simulink model "u2i_4"  (R2024a)
settings: Solver=VariableStepAuto  StartTime=0.0  StopTime=0.1  RelTol=1e-3
libraries: fl_lib x107, ee_lib x90, nesl_utility x40
(part 1 of 9)
settings Model: Creator=ltnbda  LastModifiedBy=dbagn
settings RTWCC: GPUComputeCapability=3.5

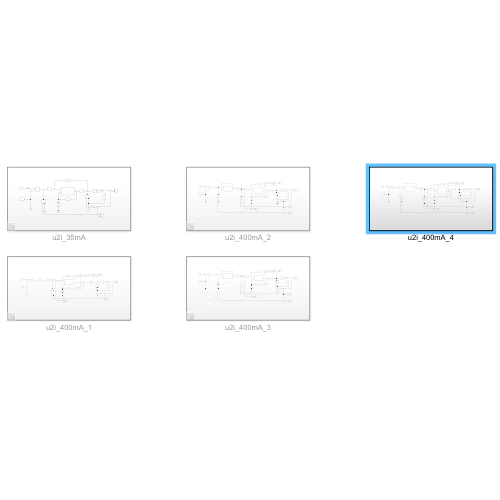
[thumbnail: Simulink's stored preview of the top-level diagram]
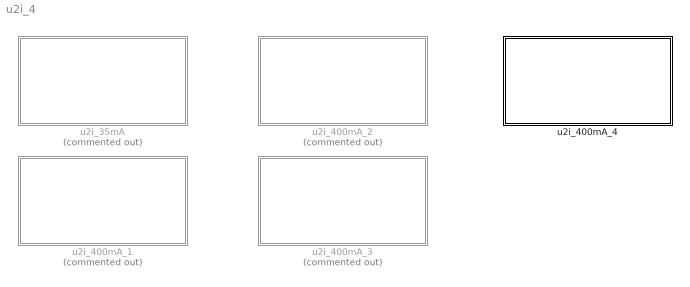
== system u2i_4 ==
  u2i_35mA : Subsystem  Commented=on
  u2i_400mA_1 : Subsystem  Commented=on
  u2i_400mA_2 : Subsystem  Commented=on
  u2i_400mA_3 : Subsystem  Commented=on
  u2i_400mA_4 : Subsystem

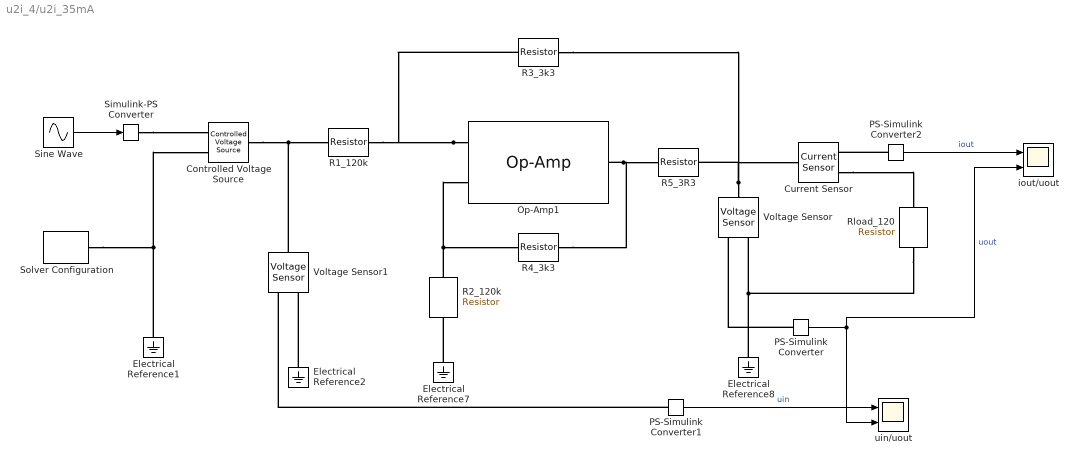
== system u2i_4/u2i_35mA ==
  Controlled Voltage Source : fl_lib/Electrical/Electrical Sources/Controlled Voltage Source
  Current Sensor : fl_lib/Electrical/Electrical Sensors/Current Sensor
  Electrical Reference{1..2,7..8} (4 alike) : fl_lib/Electrical/Electrical Elements/Electrical Reference
  Op-Amp1 : fl_lib/Electrical/Electrical Elements/Op-Amp  outI_specify=off  outI_priority=None  outI=0 A  outI_nominal_specify=off  outI_nominal_value=1  outI_nominal_unit=A
  PS-Simulink Converter : nesl_utility/PS-Simulink Converter  PhysicalDomain=network_engine_domain  SubClassName=ps_output  LeftPortType=input  RightPortType=output  PseudoPeriodic=off  Frequencies=[]  VectorFormat=1-D array  Unit=V  AffineConversion=off
  PS-Simulink Converter1 : nesl_utility/PS-Simulink Converter  PhysicalDomain=network_engine_domain  SubClassName=ps_output  LeftPortType=input  RightPortType=output  PseudoPeriodic=off  Frequencies=[]  VectorFormat=1-D array  Unit=V  AffineConversion=off
  PS-Simulink Converter2 : nesl_utility/PS-Simulink Converter  PhysicalDomain=network_engine_domain  SubClassName=ps_output  LeftPortType=input  RightPortType=output  PseudoPeriodic=off  Frequencies=[]  VectorFormat=1-D array  Unit=A  AffineConversion=off
  R1_120k : fl_lib/Electrical/Electrical Elements/Resistor  R=120e3 Ohm  i_specify=off  i_priority=None  i=0 A  i_nominal_specify=off  i_nominal_value=1  i_nominal_unit=A  v_specify=off  v_priority=None  v=0 V  v_nominal_specify=off  v_nominal_value=1  v_nominal_unit=V
  R2_120k : fl_lib/Electrical/Electrical Elements/Resistor  R=120e3 Ohm  i_specify=off  i_priority=None  i=0 A  i_nominal_specify=off  i_nominal_value=1  i_nominal_unit=A  v_specify=off  v_priority=None  v=0 V  v_nominal_specify=off  v_nominal_value=1  v_nominal_unit=V
  R3_3k3 : fl_lib/Electrical/Electrical Elements/Resistor  R=3.3e3 Ohm  i_specify=off  i_priority=None  i=0 A  i_nominal_specify=off  i_nominal_value=1  i_nominal_unit=A  v_specify=off  v_priority=None  v=0 V  v_nominal_specify=off  v_nominal_value=1  v_nominal_unit=V
  R4_3k3 : fl_lib/Electrical/Electrical Elements/Resistor  R=3.3e3 Ohm  i_specify=off  i_priority=None  i=0 A  i_nominal_specify=off  i_nominal_value=1  i_nominal_unit=A  v_specify=off  v_priority=None  v=0 V  v_nominal_specify=off  v_nominal_value=1  v_nominal_unit=V
  R5_3R3 : fl_lib/Electrical/Electrical Elements/Resistor  R=3.3 Ohm  i_specify=off  i_priority=None  i=0 A  i_nominal_specify=off  i_nominal_value=1  i_nominal_unit=A  v_specify=off  v_priority=None  v=0 V  v_nominal_specify=off  v_nominal_value=1  v_nominal_unit=V
  Rload_120 : fl_lib/Electrical/Electrical Elements/Resistor  R=12 Ohm  i_specify=off  i_priority=None  i=0 A  i_nominal_specify=off  i_nominal_value=1  i_nominal_unit=A  v_specify=off  v_priority=None  v=0 V  v_nominal_specify=off  v_nominal_value=1  v_nominal_unit=V
  Simulink-PS Converter : nesl_utility/Simulink-PS Converter  PhysicalDomain=network_engine_domain  SubClassName=ps_input  LeftPortType=input  RightPortType=output  PseudoPeriodic=off  Frequencies=[]  NoiseDistribution=none  NoiseParameters=[]  Unit=V  AffineConversion=off  FilteringAndDerivatives=provide  SimscapeFilterOrder=1  InputFilterTimeConstant=0.001  UdotUserProvided=0
  Sine Wave : Sin  Amplitude=2  Frequency=2*pi*50  SampleTime=0
  Solver Configuration : nesl_utility/Solver Configuration  PhysicalDomain=network_engine_domain  SubClassName=solver  LeftPortType=input  RightPortType=generic  Tones=[]  Harmonics=[]  SimulateNoise=off  Profile=off  UseLocalSampling=off  EnableSwitchedLinearOptims=on  FrequencyDomain=off  UseCCode=off  RelTol=0.001  AbsTol=0.001  MinStep=1e-09  ToWorkspace=off  RevertToSquareIcSolve=off  NumHomotopyIterations=100  PhasorMode=off  PhasorModeNumHarmonics=1  ConsistencySolver=NEWTON_XTOL_AFTER_FTOL  IndexReductionMethod=DerivativeReplacement  DoDC=on  ResidualTolerance=1e-09  ConsistencyTolSource=GLOBAL  ConsistencyAbsTol=0.001  ConsistencyRelTol=0.001  ConsistencyTolFactor=0.001  UseLocalSolver=on  LocalSolverChoice=NE_BACKWARD_EULER_ADVANCER  ResolveIndetEquations=on  FunctionEvalNumThread=1  LocalSolverSampleTime=1e-6  DoFixedCost=on  MaxNonlinIter=3  MaxModeIter=2  ComputeImpulses=off  ImpulseIterations=2  LinearAlgebra=auto  LinearAlgebraNumThread=0  EquationFormulation=NE_TIME_EF  DelaysMemoryBudget=1024  AutomaticFiltering=on  FilteringTimeConstant=0.001  PartitionStorageMethod=AS_NEEDED  PartitionMemoryBudget=1024  PartitionMethod=ROBUST  MultibodyUseLocalSolver=off  MultibodyLocalSolverChoice=ODE1  MultibodyLocalSolverSampleTime=0.001
  Voltage Sensor : fl_lib/Electrical/Electrical Sensors/Voltage Sensor
  Voltage Sensor1 : fl_lib/Electrical/Electrical Sensors/Voltage Sensor
  iout/uout : Scope  NumInputPorts=2
  uin/uout : Scope  NumInputPorts=2
  wires:
  PS-Simulink Converter2/1 -> iout/uout/1  "iout"
  PS-Simulink Converter1/1 -> uin/uout/1  "uin"
  PS-Simulink Converter/1 -> uin/uout/2, iout/uout/2  "uout"
  Sine Wave/1 -> Simulink-PS Converter/1
  connections:
  Voltage Sensor/LConn1 -- Current Sensor/LConn1 -- R3_3k3/RConn1 -- R5_3R3/RConn1
  Op-Amp1/RConn1 -- R5_3R3/LConn1 -- R4_3k3/RConn1
  R2_120k/LConn1 -- R4_3k3/LConn1 -- Op-Amp1/LConn2
  Electrical Reference8/LConn1 -- Voltage Sensor/RConn2 -- Rload_120/RConn1
  Electrical Reference1/LConn1 -- Solver Configuration/RConn1 -- Controlled Voltage Source/RConn2
  Op-Amp1/LConn1 -- R3_3k3/LConn1 -- R1_120k/RConn1
  PS-Simulink Converter/LConn1 -- Voltage Sensor/RConn1
  Electrical Reference7/LConn1 -- R2_120k/RConn1
  Simulink-PS Converter/RConn1 -- Controlled Voltage Source/RConn1
  Electrical Reference2/LConn1 -- Voltage Sensor1/RConn2
  Controlled Voltage Source/LConn1 -- Voltage Sensor1/LConn1 -- R1_120k/LConn1
  PS-Simulink Converter2/LConn1 -- Current Sensor/RConn1
  Current Sensor/RConn2 -- Rload_120/LConn1
  PS-Simulink Converter1/LConn1 -- Voltage Sensor1/RConn1

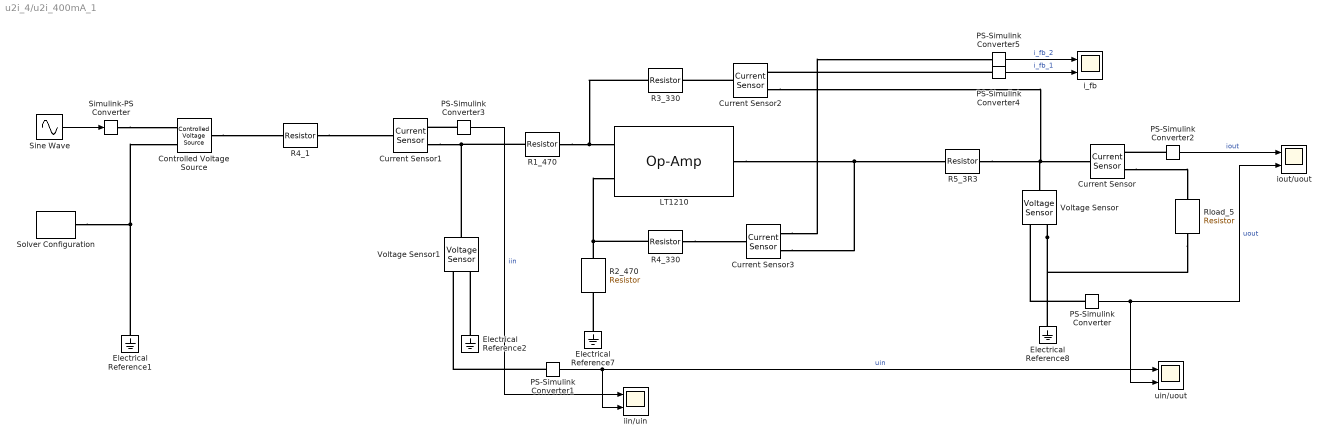
== system u2i_4/u2i_400mA_1 ==
  Controlled Voltage Source : fl_lib/Electrical/Electrical Sources/Controlled Voltage Source
  Current Sensor{,1..3} (4 alike) : fl_lib/Electrical/Electrical Sensors/Current Sensor
  Electrical Reference{1..2,7..8} (4 alike) : fl_lib/Electrical/Electrical Elements/Electrical Reference
  LT1210 : fl_lib/Electrical/Electrical Elements/Op-Amp  outI_specify=off  outI_priority=None  outI=0 A  outI_nominal_specify=off  outI_nominal_value=1  outI_nominal_unit=A
  PS-Simulink Converter : nesl_utility/PS-Simulink Converter  PhysicalDomain=network_engine_domain  SubClassName=ps_output  LeftPortType=input  RightPortType=output  PseudoPeriodic=off  Frequencies=[]  VectorFormat=1-D array  Unit=V  AffineConversion=off
  PS-Simulink Converter1 : nesl_utility/PS-Simulink Converter  PhysicalDomain=network_engine_domain  SubClassName=ps_output  LeftPortType=input  RightPortType=output  PseudoPeriodic=off  Frequencies=[]  VectorFormat=1-D array  Unit=V  AffineConversion=off
  PS-Simulink Converter{2..5} (4 alike) : nesl_utility/PS-Simulink Converter  PhysicalDomain=network_engine_domain  SubClassName=ps_output  LeftPortType=input  RightPortType=output  PseudoPeriodic=off  Frequencies=[]  VectorFormat=1-D array  Unit=A  AffineConversion=off
  R1_470 : fl_lib/Electrical/Electrical Elements/Resistor  R=470 Ohm  i_specify=off  i_priority=None  i=0 A  i_nominal_specify=off  i_nominal_value=1  i_nominal_unit=A  v_specify=off  v_priority=None  v=0 V  v_nominal_specify=off  v_nominal_value=1  v_nominal_unit=V
  R2_470 : fl_lib/Electrical/Electrical Elements/Resistor  R=470 Ohm  i_specify=off  i_priority=None  i=0 A  i_nominal_specify=off  i_nominal_value=1  i_nominal_unit=A  v_specify=off  v_priority=None  v=0 V  v_nominal_specify=off  v_nominal_value=1  v_nominal_unit=V
  R3_330 : fl_lib/Electrical/Electrical Elements/Resistor  R=330 Ohm  i_specify=off  i_priority=None  i=0 A  i_nominal_specify=off  i_nominal_value=1  i_nominal_unit=A  v_specify=off  v_priority=None  v=0 V  v_nominal_specify=off  v_nominal_value=1  v_nominal_unit=V
  R4_1 : fl_lib/Electrical/Electrical Elements/Resistor  R=0 Ohm  i_specify=off  i_priority=None  i=0 A  i_nominal_specify=off  i_nominal_value=1  i_nominal_unit=A  v_specify=off  v_priority=None  v=0 V  v_nominal_specify=off  v_nominal_value=1  v_nominal_unit=V
  R4_330 : fl_lib/Electrical/Electrical Elements/Resistor  R=330 Ohm  i_specify=off  i_priority=None  i=0 A  i_nominal_specify=off  i_nominal_value=1  i_nominal_unit=A  v_specify=off  v_priority=None  v=0 V  v_nominal_specify=off  v_nominal_value=1  v_nominal_unit=V
  R5_3R3 : fl_lib/Electrical/Electrical Elements/Resistor  R=3.3 Ohm  i_specify=off  i_priority=None  i=0 A  i_nominal_specify=off  i_nominal_value=1  i_nominal_unit=A  v_specify=off  v_priority=None  v=0 V  v_nominal_specify=off  v_nominal_value=1  v_nominal_unit=V
  Rload_5 : fl_lib/Electrical/Electrical Elements/Resistor  R=10 Ohm  i_specify=off  i_priority=None  i=0 A  i_nominal_specify=off  i_nominal_value=1  i_nominal_unit=A  v_specify=off  v_priority=None  v=0 V  v_nominal_specify=off  v_nominal_value=1  v_nominal_unit=V
  Simulink-PS Converter : nesl_utility/Simulink-PS Converter  PhysicalDomain=network_engine_domain  SubClassName=ps_input  LeftPortType=input  RightPortType=output  PseudoPeriodic=off  Frequencies=[]  NoiseDistribution=none  NoiseParameters=[]  Unit=V  AffineConversion=off  FilteringAndDerivatives=provide  SimscapeFilterOrder=1  InputFilterTimeConstant=0.001  UdotUserProvided=0
  Sine Wave : Sin  Amplitude=2  Frequency=2*pi*50  SampleTime=0
  Solver Configuration : nesl_utility/Solver Configuration  PhysicalDomain=network_engine_domain  SubClassName=solver  LeftPortType=input  RightPortType=generic  Tones=[]  Harmonics=[]  SimulateNoise=off  Profile=off  UseLocalSampling=off  EnableSwitchedLinearOptims=on  FrequencyDomain=off  UseCCode=off  RelTol=0.001  AbsTol=0.001  MinStep=1e-09  ToWorkspace=off  RevertToSquareIcSolve=off  NumHomotopyIterations=100  PhasorMode=off  PhasorModeNumHarmonics=1  ConsistencySolver=NEWTON_XTOL_AFTER_FTOL  IndexReductionMethod=DerivativeReplacement  DoDC=on  ResidualTolerance=1e-09  ConsistencyTolSource=GLOBAL  ConsistencyAbsTol=0.001  ConsistencyRelTol=0.001  ConsistencyTolFactor=0.001  UseLocalSolver=on  LocalSolverChoice=NE_BACKWARD_EULER_ADVANCER  ResolveIndetEquations=on  FunctionEvalNumThread=1  LocalSolverSampleTime=1e-6  DoFixedCost=on  MaxNonlinIter=3  MaxModeIter=2  ComputeImpulses=off  ImpulseIterations=2  LinearAlgebra=auto  LinearAlgebraNumThread=0  EquationFormulation=NE_TIME_EF  DelaysMemoryBudget=1024  AutomaticFiltering=on  FilteringTimeConstant=0.001  PartitionStorageMethod=AS_NEEDED  PartitionMemoryBudget=1024  PartitionMethod=ROBUST  MultibodyUseLocalSolver=off  MultibodyLocalSolverChoice=ODE1  MultibodyLocalSolverSampleTime=0.001
  Voltage Sensor : fl_lib/Electrical/Electrical Sensors/Voltage Sensor
  Voltage Sensor1 : fl_lib/Electrical/Electrical Sensors/Voltage Sensor
  i_fb : Scope  NumInputPorts=2
  iin/uin : Scope  NumInputPorts=2
  iout/uout : Scope  NumInputPorts=2
  uin/uout : Scope  NumInputPorts=2
  wires:
  Sine Wave/1 -> Simulink-PS Converter/1
  PS-Simulink Converter/1 -> iout/uout/2, uin/uout/2  "uout"
  PS-Simulink Converter1/1 -> uin/uout/1, iin/uin/2  "uin"
  PS-Simulink Converter2/1 -> iout/uout/1  "iout"
  PS-Simulink Converter3/1 -> iin/uin/1  "iin"
  PS-Simulink Converter4/1 -> i_fb/2  "i_fb_1"
  PS-Simulink Converter5/1 -> i_fb/1  "i_fb_2"
  connections:
  PS-Simulink Converter1/LConn1 -- Voltage Sensor1/RConn1
  Current Sensor/RConn2 -- Rload_5/LConn1
  PS-Simulink Converter2/LConn1 -- Current Sensor/RConn1
  Voltage Sensor1/LConn1 -- R1_470/LConn1 -- Current Sensor1/RConn2
  Electrical Reference2/LConn1 -- Voltage Sensor1/RConn2
  Simulink-PS Converter/RConn1 -- Controlled Voltage Source/RConn1
  Electrical Reference7/LConn1 -- R2_470/RConn1
  PS-Simulink Converter/LConn1 -- Voltage Sensor/RConn1
  Solver Configuration/RConn1 -- Controlled Voltage Source/RConn2 -- Electrical Reference1/LConn1
  Voltage Sensor/RConn2 -- Electrical Reference8/LConn1 -- Rload_5/RConn1
  R2_470/LConn1 -- LT1210/LConn2 -- R4_330/LConn1
  LT1210/RConn1 -- Current Sensor3/RConn2 -- R5_3R3/LConn1
  PS-Simulink Converter3/LConn1 -- Current Sensor1/RConn1
  R1_470/RConn1 -- R3_330/LConn1 -- LT1210/LConn1
  R5_3R3/RConn1 -- Current Sensor2/RConn2 -- Voltage Sensor/LConn1 -- Current Sensor/LConn1
  R4_1/RConn1 -- Current Sensor1/LConn1
  Current Sensor2/LConn1 -- R3_330/RConn1
  PS-Simulink Converter4/LConn1 -- Current Sensor2/RConn1
  R4_330/RConn1 -- Current Sensor3/LConn1
  Current Sensor3/RConn1 -- PS-Simulink Converter5/LConn1
  Controlled Voltage Source/LConn1 -- R4_1/LConn1

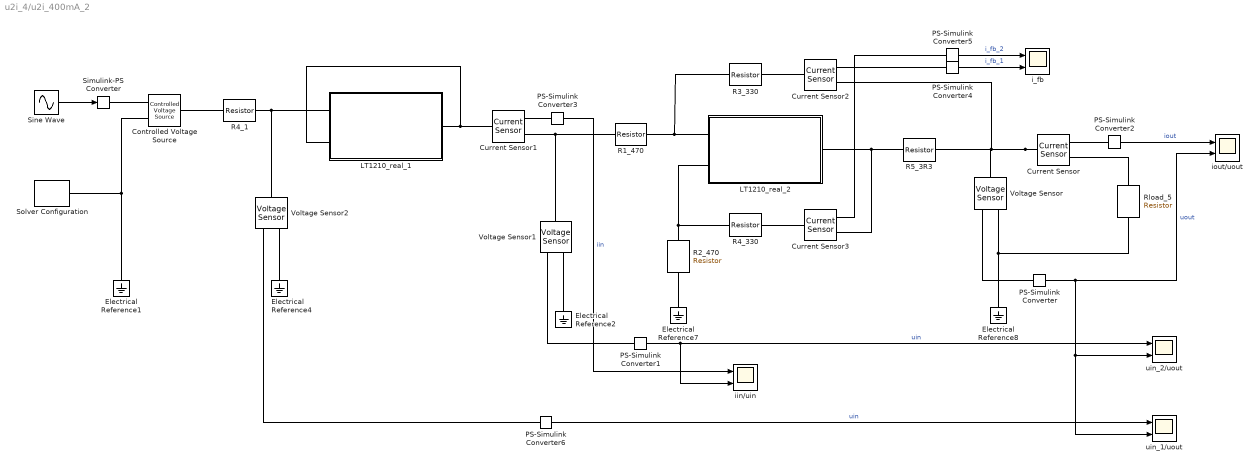
== system u2i_4/u2i_400mA_2 ==
  Controlled Voltage Source : fl_lib/Electrical/Electrical Sources/Controlled Voltage Source
  Current Sensor{,1..3} (4 alike) : fl_lib/Electrical/Electrical Sensors/Current Sensor
  Electrical Reference{1..2,4,7..8} (5 alike) : fl_lib/Electrical/Electrical Elements/Electrical Reference
  LT1210_real_1 : Subsystem
  LT1210_real_2 : Subsystem
  PS-Simulink Converter : nesl_utility/PS-Simulink Converter  PhysicalDomain=network_engine_domain  SubClassName=ps_output  LeftPortType=input  RightPortType=output  PseudoPeriodic=off  Frequencies=[]  VectorFormat=1-D array  Unit=V  AffineConversion=off
  PS-Simulink Converter1 : nesl_utility/PS-Simulink Converter  PhysicalDomain=network_engine_domain  SubClassName=ps_output  LeftPortType=input  RightPortType=output  PseudoPeriodic=off  Frequencies=[]  VectorFormat=1-D array  Unit=V  AffineConversion=off
  PS-Simulink Converter{2..5} (4 alike) : nesl_utility/PS-Simulink Converter  PhysicalDomain=network_engine_domain  SubClassName=ps_output  LeftPortType=input  RightPortType=output  PseudoPeriodic=off  Frequencies=[]  VectorFormat=1-D array  Unit=A  AffineConversion=off
  PS-Simulink Converter6 : nesl_utility/PS-Simulink Converter  PhysicalDomain=network_engine_domain  SubClassName=ps_output  LeftPortType=input  RightPortType=output  PseudoPeriodic=off  Frequencies=[]  VectorFormat=1-D array  Unit=V  AffineConversion=off
  R1_470 : fl_lib/Electrical/Electrical Elements/Resistor  R=470 Ohm  i_specify=off  i_priority=None  i=0 A  i_nominal_specify=off  i_nominal_value=1  i_nominal_unit=A  v_specify=off  v_priority=None  v=0 V  v_nominal_specify=off  v_nominal_value=1  v_nominal_unit=V
  R2_470 : fl_lib/Electrical/Electrical Elements/Resistor  R=470 Ohm  i_specify=off  i_priority=None  i=0 A  i_nominal_specify=off  i_nominal_value=1  i_nominal_unit=A  v_specify=off  v_priority=None  v=0 V  v_nominal_specify=off  v_nominal_value=1  v_nominal_unit=V
  R3_330 : fl_lib/Electrical/Electrical Elements/Resistor  R=330 Ohm  i_specify=off  i_priority=None  i=0 A  i_nominal_specify=off  i_nominal_value=1  i_nominal_unit=A  v_specify=off  v_priority=None  v=0 V  v_nominal_specify=off  v_nominal_value=1  v_nominal_unit=V
  R4_1 : fl_lib/Electrical/Electrical Elements/Resistor  R=1e3 Ohm  i_specify=off  i_priority=None  i=0 A  i_nominal_specify=off  i_nominal_value=1  i_nominal_unit=A  v_specify=off  v_priority=None  v=0 V  v_nominal_specify=off  v_nominal_value=1  v_nominal_unit=V
  R4_330 : fl_lib/Electrical/Electrical Elements/Resistor  R=330 Ohm  i_specify=off  i_priority=None  i=0 A  i_nominal_specify=off  i_nominal_value=1  i_nominal_unit=A  v_specify=off  v_priority=None  v=0 V  v_nominal_specify=off  v_nominal_value=1  v_nominal_unit=V
  R5_3R3 : fl_lib/Electrical/Electrical Elements/Resistor  R=3.3 Ohm  i_specify=off  i_priority=None  i=0 A  i_nominal_specify=off  i_nominal_value=1  i_nominal_unit=A  v_specify=off  v_priority=None  v=0 V  v_nominal_specify=off  v_nominal_value=1  v_nominal_unit=V
  Rload_5 : fl_lib/Electrical/Electrical Elements/Resistor  R=10 Ohm  i_specify=off  i_priority=None  i=0 A  i_nominal_specify=off  i_nominal_value=1  i_nominal_unit=A  v_specify=off  v_priority=None  v=0 V  v_nominal_specify=off  v_nominal_value=1  v_nominal_unit=V
  Simulink-PS Converter : nesl_utility/Simulink-PS Converter  PhysicalDomain=network_engine_domain  SubClassName=ps_input  LeftPortType=input  RightPortType=output  PseudoPeriodic=off  Frequencies=[]  NoiseDistribution=none  NoiseParameters=[]  Unit=V  AffineConversion=off  FilteringAndDerivatives=provide  SimscapeFilterOrder=1  InputFilterTimeConstant=0.001  UdotUserProvided=0
  Sine Wave : Sin  Amplitude=2  Frequency=2*pi*50  SampleTime=0
  Solver Configuration : nesl_utility/Solver Configuration  PhysicalDomain=network_engine_domain  SubClassName=solver  LeftPortType=input  RightPortType=generic  Tones=[]  Harmonics=[]  SimulateNoise=off  Profile=off  UseLocalSampling=off  EnableSwitchedLinearOptims=on  FrequencyDomain=off  UseCCode=off  RelTol=0.001  AbsTol=0.001  MinStep=1e-09  ToWorkspace=off  RevertToSquareIcSolve=off  NumHomotopyIterations=100  PhasorMode=off  PhasorModeNumHarmonics=1  ConsistencySolver=NEWTON_XTOL_AFTER_FTOL  IndexReductionMethod=DerivativeReplacement  DoDC=on  ResidualTolerance=1e-09  ConsistencyTolSource=GLOBAL  ConsistencyAbsTol=0.001  ConsistencyRelTol=0.001  ConsistencyTolFactor=0.001  UseLocalSolver=on  LocalSolverChoice=NE_BACKWARD_EULER_ADVANCER  ResolveIndetEquations=on  FunctionEvalNumThread=1  LocalSolverSampleTime=1e-6  DoFixedCost=on  MaxNonlinIter=3  MaxModeIter=2  ComputeImpulses=off  ImpulseIterations=2  LinearAlgebra=auto  LinearAlgebraNumThread=0  EquationFormulation=NE_TIME_EF  DelaysMemoryBudget=1024  AutomaticFiltering=on  FilteringTimeConstant=0.001  PartitionStorageMethod=AS_NEEDED  PartitionMemoryBudget=1024  PartitionMethod=ROBUST  MultibodyUseLocalSolver=off  MultibodyLocalSolverChoice=ODE1  MultibodyLocalSolverSampleTime=0.001
  Voltage Sensor : fl_lib/Electrical/Electrical Sensors/Voltage Sensor
  Voltage Sensor1 : fl_lib/Electrical/Electrical Sensors/Voltage Sensor
  Voltage Sensor2 : fl_lib/Electrical/Electrical Sensors/Voltage Sensor
  i_fb : Scope  NumInputPorts=2
  iin/uin : Scope  NumInputPorts=2
  iout/uout : Scope  NumInputPorts=2
  uin_1/uout : Scope  NumInputPorts=2
  uin_2/uout : Scope  NumInputPorts=2
  wires:
  PS-Simulink Converter5/1 -> i_fb/1  "i_fb_2"
  PS-Simulink Converter4/1 -> i_fb/2  "i_fb_1"
  PS-Simulink Converter3/1 -> iin/uin/1  "iin"
  PS-Simulink Converter2/1 -> iout/uout/1  "iout"
  PS-Simulink Converter1/1 -> uin_2/uout/1, iin/uin/2  "uin"
  PS-Simulink Converter/1 -> uin_1/uout/2, uin_2/uout/2, iout/uout/2  "uout"
  Sine Wave/1 -> Simulink-PS Converter/1
  PS-Simulink Converter6/1 -> uin_1/uout/1  "uin"
  connections:
  Controlled Voltage Source/LConn1 -- R4_1/LConn1
  Current Sensor3/RConn1 -- PS-Simulink Converter5/LConn1
  R4_330/RConn1 -- Current Sensor3/LConn1
  PS-Simulink Converter4/LConn1 -- Current Sensor2/RConn1
  Current Sensor2/LConn1 -- R3_330/RConn1
  Current Sensor/LConn1 -- R5_3R3/RConn1 -- Voltage Sensor/LConn1 -- Current Sensor2/RConn2
  R3_330/LConn1 -- LT1210_real_2/LConn1 -- R1_470/RConn1
  PS-Simulink Converter3/LConn1 -- Current Sensor1/RConn1
  Current Sensor3/RConn2 -- LT1210_real_2/RConn1 -- R5_3R3/LConn1
  R4_330/LConn1 -- LT1210_real_2/LConn2 -- R2_470/LConn1
  Rload_5/RConn1 -- Electrical Reference8/LConn1 -- Voltage Sensor/RConn2
  Electrical Reference1/LConn1 -- Controlled Voltage Source/RConn2 -- Solver Configuration/RConn1
  PS-Simulink Converter/LConn1 -- Voltage Sensor/RConn1
  Electrical Reference7/LConn1 -- R2_470/RConn1
  Simulink-PS Converter/RConn1 -- Controlled Voltage Source/RConn1
  Electrical Reference2/LConn1 -- Voltage Sensor1/RConn2
  R1_470/LConn1 -- Voltage Sensor1/LConn1 -- Current Sensor1/RConn2
  PS-Simulink Converter2/LConn1 -- Current Sensor/RConn1
  Current Sensor/RConn2 -- Rload_5/LConn1
  PS-Simulink Converter1/LConn1 -- Voltage Sensor1/RConn1
  Voltage Sensor2/LConn1 -- LT1210_real_1/LConn1 -- R4_1/RConn1
  PS-Simulink Converter6/LConn1 -- Voltage Sensor2/RConn1
  Electrical Reference4/LConn1 -- Voltage Sensor2/RConn2
  LT1210_real_1/RConn1 -- Current Sensor1/LConn1 -- LT1210_real_1/LConn2

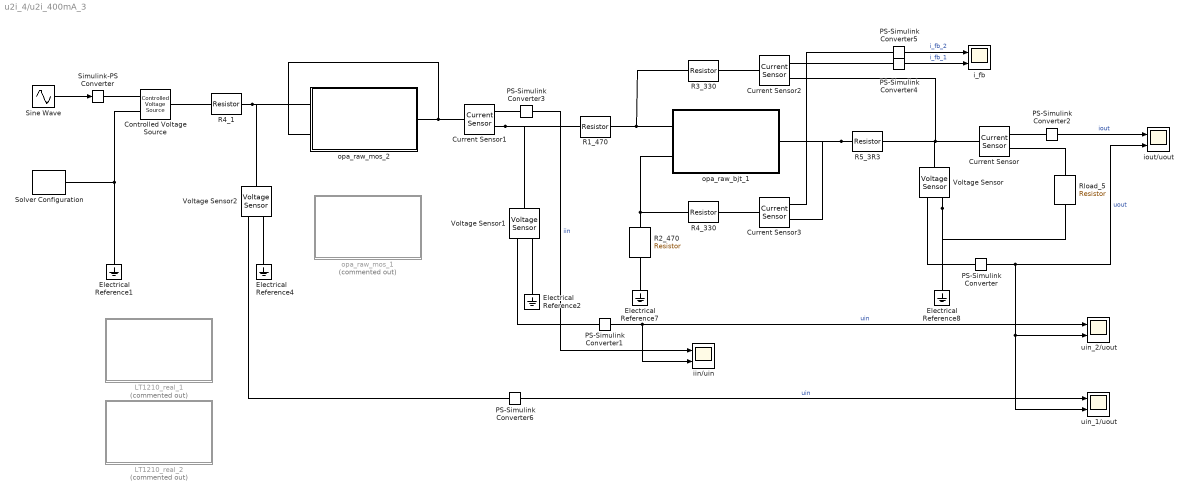
== system u2i_4/u2i_400mA_3 ==
  Controlled Voltage Source : fl_lib/Electrical/Electrical Sources/Controlled Voltage Source
  Current Sensor{,1..3} (4 alike) : fl_lib/Electrical/Electrical Sensors/Current Sensor
  Electrical Reference{1..2,4,7..8} (5 alike) : fl_lib/Electrical/Electrical Elements/Electrical Reference
  LT1210_real_1 : Subsystem  Commented=on
  LT1210_real_2 : Subsystem  Commented=on
  PS-Simulink Converter : nesl_utility/PS-Simulink Converter  PhysicalDomain=network_engine_domain  SubClassName=ps_output  LeftPortType=input  RightPortType=output  PseudoPeriodic=off  Frequencies=[]  VectorFormat=1-D array  Unit=V  AffineConversion=off
  PS-Simulink Converter1 : nesl_utility/PS-Simulink Converter  PhysicalDomain=network_engine_domain  SubClassName=ps_output  LeftPortType=input  RightPortType=output  PseudoPeriodic=off  Frequencies=[]  VectorFormat=1-D array  Unit=V  AffineConversion=off
  PS-Simulink Converter{2..5} (4 alike) : nesl_utility/PS-Simulink Converter  PhysicalDomain=network_engine_domain  SubClassName=ps_output  LeftPortType=input  RightPortType=output  PseudoPeriodic=off  Frequencies=[]  VectorFormat=1-D array  Unit=A  AffineConversion=off
  PS-Simulink Converter6 : nesl_utility/PS-Simulink Converter  PhysicalDomain=network_engine_domain  SubClassName=ps_output  LeftPortType=input  RightPortType=output  PseudoPeriodic=off  Frequencies=[]  VectorFormat=1-D array  Unit=V  AffineConversion=off
  R1_470 : fl_lib/Electrical/Electrical Elements/Resistor  R=470 Ohm  i_specify=off  i_priority=None  i=0 A  i_nominal_specify=off  i_nominal_value=1  i_nominal_unit=A  v_specify=off  v_priority=None  v=0 V  v_nominal_specify=off  v_nominal_value=1  v_nominal_unit=V
  R2_470 : fl_lib/Electrical/Electrical Elements/Resistor  R=470 Ohm  i_specify=off  i_priority=None  i=0 A  i_nominal_specify=off  i_nominal_value=1  i_nominal_unit=A  v_specify=off  v_priority=None  v=0 V  v_nominal_specify=off  v_nominal_value=1  v_nominal_unit=V
  R3_330 : fl_lib/Electrical/Electrical Elements/Resistor  R=330 Ohm  i_specify=off  i_priority=None  i=0 A  i_nominal_specify=off  i_nominal_value=1  i_nominal_unit=A  v_specify=off  v_priority=None  v=0 V  v_nominal_specify=off  v_nominal_value=1  v_nominal_unit=V
  R4_1 : fl_lib/Electrical/Electrical Elements/Resistor  R=1e3 Ohm  i_specify=off  i_priority=None  i=0 A  i_nominal_specify=off  i_nominal_value=1  i_nominal_unit=A  v_specify=off  v_priority=None  v=0 V  v_nominal_specify=off  v_nominal_value=1  v_nominal_unit=V
  R4_330 : fl_lib/Electrical/Electrical Elements/Resistor  R=330 Ohm  i_specify=off  i_priority=None  i=0 A  i_nominal_specify=off  i_nominal_value=1  i_nominal_unit=A  v_specify=off  v_priority=None  v=0 V  v_nominal_specify=off  v_nominal_value=1  v_nominal_unit=V
  R5_3R3 : fl_lib/Electrical/Electrical Elements/Resistor  R=3.3 Ohm  i_specify=off  i_priority=None  i=0 A  i_nominal_specify=off  i_nominal_value=1  i_nominal_unit=A  v_specify=off  v_priority=None  v=0 V  v_nominal_specify=off  v_nominal_value=1  v_nominal_unit=V
  Rload_5 : fl_lib/Electrical/Electrical Elements/Resistor  R=5 Ohm  i_specify=off  i_priority=None  i=0 A  i_nominal_specify=off  i_nominal_value=1  i_nominal_unit=A  v_specify=off  v_priority=None  v=0 V  v_nominal_specify=off  v_nominal_value=1  v_nominal_unit=V
  Simulink-PS Converter : nesl_utility/Simulink-PS Converter  PhysicalDomain=network_engine_domain  SubClassName=ps_input  LeftPortType=input  RightPortType=output  PseudoPeriodic=off  Frequencies=[]  NoiseDistribution=none  NoiseParameters=[]  Unit=V  AffineConversion=off  FilteringAndDerivatives=provide  SimscapeFilterOrder=1  InputFilterTimeConstant=0.001  UdotUserProvided=0
  Sine Wave : Sin  Amplitude=2  Frequency=2*pi*50  SampleTime=0
  Solver Configuration : nesl_utility/Solver Configuration  PhysicalDomain=network_engine_domain  SubClassName=solver  LeftPortType=input  RightPortType=generic  Tones=[]  Harmonics=[]  SimulateNoise=off  Profile=off  UseLocalSampling=off  EnableSwitchedLinearOptims=on  FrequencyDomain=off  UseCCode=off  RelTol=0.001  AbsTol=0.001  MinStep=1e-09  ToWorkspace=off  RevertToSquareIcSolve=off  NumHomotopyIterations=100  PhasorMode=off  PhasorModeNumHarmonics=1  ConsistencySolver=NEWTON_XTOL_AFTER_FTOL  IndexReductionMethod=DerivativeReplacement  DoDC=on  ResidualTolerance=1e-09  ConsistencyTolSource=GLOBAL  ConsistencyAbsTol=0.001  ConsistencyRelTol=0.001  ConsistencyTolFactor=0.001  UseLocalSolver=on  LocalSolverChoice=NE_BACKWARD_EULER_ADVANCER  ResolveIndetEquations=on  FunctionEvalNumThread=1  LocalSolverSampleTime=1e-6  DoFixedCost=on  MaxNonlinIter=3  MaxModeIter=2  ComputeImpulses=off  ImpulseIterations=2  LinearAlgebra=auto  LinearAlgebraNumThread=0  EquationFormulation=NE_TIME_EF  DelaysMemoryBudget=1024  AutomaticFiltering=on  FilteringTimeConstant=0.001  PartitionStorageMethod=AS_NEEDED  PartitionMemoryBudget=1024  PartitionMethod=ROBUST  MultibodyUseLocalSolver=off  MultibodyLocalSolverChoice=ODE1  MultibodyLocalSolverSampleTime=0.001
  Voltage Sensor : fl_lib/Electrical/Electrical Sensors/Voltage Sensor
  Voltage Sensor1 : fl_lib/Electrical/Electrical Sensors/Voltage Sensor
  Voltage Sensor2 : fl_lib/Electrical/Electrical Sensors/Voltage Sensor
  i_fb : Scope  NumInputPorts=2
  iin/uin : Scope  NumInputPorts=2
  iout/uout : Scope  NumInputPorts=2
  opa_raw_bjt_1 : Subsystem  mask{u_dd=15, u_ss=-15, beta_f=100, Rbias=300, Ibias=1}
      mask prompts: u_dd "Udd"; u_ss "Uss"; beta_f "Betaf"
  opa_raw_mos_1 : Subsystem  Commented=on  mask{u_dd=15, u_ss=-15, Rbias=1e3, Ibias=1}
      mask prompts: u_dd "Udd"; u_ss "Uss"
  opa_raw_mos_2 : Subsystem  mask{u_dd=15, u_ss=-15, Rbias=1e3, Ibias=10e-3}
      mask prompts: u_dd "Udd"; u_ss "Uss"
  uin_1/uout : Scope  NumInputPorts=2
  uin_2/uout : Scope  NumInputPorts=2
  wires:
  PS-Simulink Converter6/1 -> uin_1/uout/1  "uin"
  Sine Wave/1 -> Simulink-PS Converter/1
  PS-Simulink Converter/1 -> iout/uout/2, uin_2/uout/2, uin_1/uout/2  "uout"
  PS-Simulink Converter1/1 -> iin/uin/2, uin_2/uout/1  "uin"
  PS-Simulink Converter2/1 -> iout/uout/1  "iout"
  PS-Simulink Converter3/1 -> iin/uin/1  "iin"
  PS-Simulink Converter4/1 -> i_fb/2  "i_fb_1"
  PS-Simulink Converter5/1 -> i_fb/1  "i_fb_2"
  connections:
  Current Sensor1/LConn1 -- opa_raw_mos_2/LConn2 -- opa_raw_mos_2/RConn1
  Electrical Reference4/LConn1 -- Voltage Sensor2/RConn2
  PS-Simulink Converter6/LConn1 -- Voltage Sensor2/RConn1
  R4_1/RConn1 -- opa_raw_mos_2/LConn1 -- Voltage Sensor2/LConn1
  PS-Simulink Converter1/LConn1 -- Voltage Sensor1/RConn1
  Current Sensor/RConn2 -- Rload_5/LConn1
  PS-Simulink Converter2/LConn1 -- Current Sensor/RConn1
  Current Sensor1/RConn2 -- Voltage Sensor1/LConn1 -- R1_470/LConn1
  Electrical Reference2/LConn1 -- Voltage Sensor1/RConn2
  Simulink-PS Converter/RConn1 -- Controlled Voltage Source/RConn1
  Electrical Reference7/LConn1 -- R2_470/RConn1
  PS-Simulink Converter/LConn1 -- Voltage Sensor/RConn1
  Solver Configuration/RConn1 -- Controlled Voltage Source/RConn2 -- Electrical Reference1/LConn1
  Voltage Sensor/RConn2 -- Electrical Reference8/LConn1 -- Rload_5/RConn1
  R2_470/LConn1 -- opa_raw_bjt_1/LConn2 -- R4_330/LConn1
  R5_3R3/LConn1 -- opa_raw_bjt_1/RConn1 -- Current Sensor3/RConn2
  PS-Simulink Converter3/LConn1 -- Current Sensor1/RConn1
  R1_470/RConn1 -- opa_raw_bjt_1/LConn1 -- R3_330/LConn1
  Current Sensor2/RConn2 -- Voltage Sensor/LConn1 -- R5_3R3/RConn1 -- Current Sensor/LConn1
  Current Sensor2/LConn1 -- R3_330/RConn1
  PS-Simulink Converter4/LConn1 -- Current Sensor2/RConn1
  R4_330/RConn1 -- Current Sensor3/LConn1
  Current Sensor3/RConn1 -- PS-Simulink Converter5/LConn1
  Controlled Voltage Source/LConn1 -- R4_1/LConn1

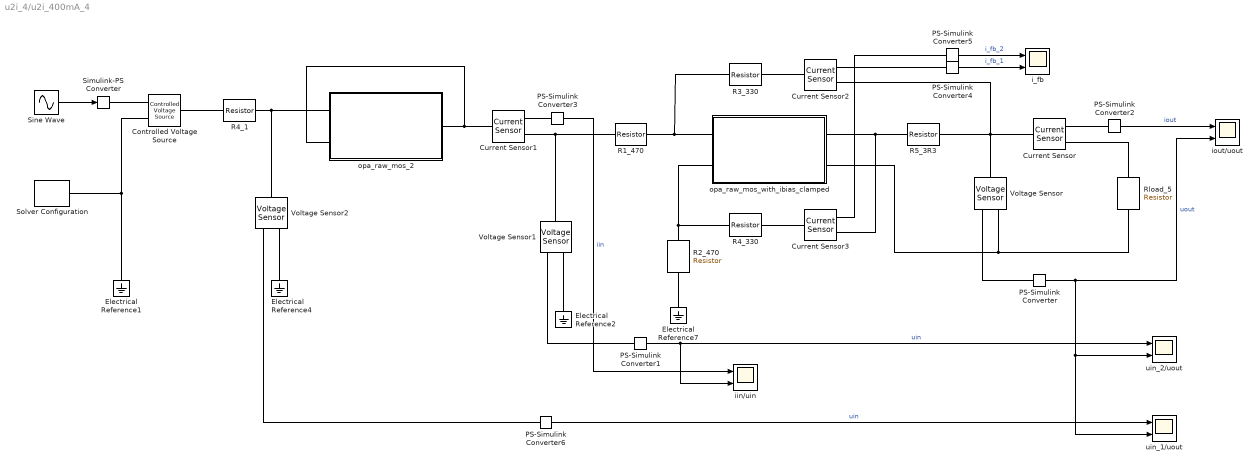
== system u2i_4/u2i_400mA_4 ==
  Controlled Voltage Source : fl_lib/Electrical/Electrical Sources/Controlled Voltage Source
  Current Sensor{,1..3} (4 alike) : fl_lib/Electrical/Electrical Sensors/Current Sensor
  Electrical Reference{1..2,4,7} (4 alike) : fl_lib/Electrical/Electrical Elements/Electrical Reference
  PS-Simulink Converter : nesl_utility/PS-Simulink Converter  PhysicalDomain=network_engine_domain  SubClassName=ps_output  LeftPortType=input  RightPortType=output  PseudoPeriodic=off  Frequencies=[]  VectorFormat=1-D array  Unit=V  AffineConversion=off
  PS-Simulink Converter1 : nesl_utility/PS-Simulink Converter  PhysicalDomain=network_engine_domain  SubClassName=ps_output  LeftPortType=input  RightPortType=output  PseudoPeriodic=off  Frequencies=[]  VectorFormat=1-D array  Unit=V  AffineConversion=off
  PS-Simulink Converter{2..5} (4 alike) : nesl_utility/PS-Simulink Converter  PhysicalDomain=network_engine_domain  SubClassName=ps_output  LeftPortType=input  RightPortType=output  PseudoPeriodic=off  Frequencies=[]  VectorFormat=1-D array  Unit=A  AffineConversion=off
  PS-Simulink Converter6 : nesl_utility/PS-Simulink Converter  PhysicalDomain=network_engine_domain  SubClassName=ps_output  LeftPortType=input  RightPortType=output  PseudoPeriodic=off  Frequencies=[]  VectorFormat=1-D array  Unit=V  AffineConversion=off
  R1_470 : fl_lib/Electrical/Electrical Elements/Resistor  R=470 Ohm  i_specify=off  i_priority=None  i=0 A  i_nominal_specify=off  i_nominal_value=1  i_nominal_unit=A  v_specify=off  v_priority=None  v=0 V  v_nominal_specify=off  v_nominal_value=1  v_nominal_unit=V
  R2_470 : fl_lib/Electrical/Electrical Elements/Resistor  R=470 Ohm  i_specify=off  i_priority=None  i=0 A  i_nominal_specify=off  i_nominal_value=1  i_nominal_unit=A  v_specify=off  v_priority=None  v=0 V  v_nominal_specify=off  v_nominal_value=1  v_nominal_unit=V
  R3_330 : fl_lib/Electrical/Electrical Elements/Resistor  R=330 Ohm  i_specify=off  i_priority=None  i=0 A  i_nominal_specify=off  i_nominal_value=1  i_nominal_unit=A  v_specify=off  v_priority=None  v=0 V  v_nominal_specify=off  v_nominal_value=1  v_nominal_unit=V
  R4_1 : fl_lib/Electrical/Electrical Elements/Resistor  R=1e3 Ohm  i_specify=off  i_priority=None  i=0 A  i_nominal_specify=off  i_nominal_value=1  i_nominal_unit=A  v_specify=off  v_priority=None  v=0 V  v_nominal_specify=off  v_nominal_value=1  v_nominal_unit=V
  R4_330 : fl_lib/Electrical/Electrical Elements/Resistor  R=330 Ohm  i_specify=off  i_priority=None  i=0 A  i_nominal_specify=off  i_nominal_value=1  i_nominal_unit=A  v_specify=off  v_priority=None  v=0 V  v_nominal_specify=off  v_nominal_value=1  v_nominal_unit=V
  R5_3R3 : fl_lib/Electrical/Electrical Elements/Resistor  R=3.3 Ohm  i_specify=off  i_priority=None  i=0 A  i_nominal_specify=off  i_nominal_value=1  i_nominal_unit=A  v_specify=off  v_priority=None  v=0 V  v_nominal_specify=off  v_nominal_value=1  v_nominal_unit=V
  Rload_5 : fl_lib/Electrical/Electrical Elements/Resistor  R=5 Ohm  i_specify=off  i_priority=None  i=0 A  i_nominal_specify=off  i_nominal_value=1  i_nominal_unit=A  v_specify=off  v_priority=None  v=0 V  v_nominal_specify=off  v_nominal_value=1  v_nominal_unit=V
  Simulink-PS Converter : nesl_utility/Simulink-PS Converter  PhysicalDomain=network_engine_domain  SubClassName=ps_input  LeftPortType=input  RightPortType=output  PseudoPeriodic=off  Frequencies=[]  NoiseDistribution=none  NoiseParameters=[]  Unit=V  AffineConversion=off  FilteringAndDerivatives=provide  SimscapeFilterOrder=1  InputFilterTimeConstant=0.001  UdotUserProvided=0
  Sine Wave : Sin  Amplitude=2  Frequency=2*pi*50  SampleTime=0
  Solver Configuration : nesl_utility/Solver Configuration  PhysicalDomain=network_engine_domain  SubClassName=solver  LeftPortType=input  RightPortType=generic  Tones=[]  Harmonics=[]  SimulateNoise=off  Profile=off  UseLocalSampling=off  EnableSwitchedLinearOptims=on  FrequencyDomain=off  UseCCode=off  RelTol=0.001  AbsTol=0.001  MinStep=1e-09  ToWorkspace=off  RevertToSquareIcSolve=off  NumHomotopyIterations=100  PhasorMode=off  PhasorModeNumHarmonics=1  ConsistencySolver=NEWTON_XTOL_AFTER_FTOL  IndexReductionMethod=DerivativeReplacement  DoDC=on  ResidualTolerance=1e-09  ConsistencyTolSource=GLOBAL  ConsistencyAbsTol=0.001  ConsistencyRelTol=0.001  ConsistencyTolFactor=0.001  UseLocalSolver=on  LocalSolverChoice=NE_BACKWARD_EULER_ADVANCER  ResolveIndetEquations=on  FunctionEvalNumThread=1  LocalSolverSampleTime=1e-6  DoFixedCost=on  MaxNonlinIter=3  MaxModeIter=2  ComputeImpulses=off  ImpulseIterations=2  LinearAlgebra=auto  LinearAlgebraNumThread=0  EquationFormulation=NE_TIME_EF  DelaysMemoryBudget=1024  AutomaticFiltering=on  FilteringTimeConstant=0.001  PartitionStorageMethod=AS_NEEDED  PartitionMemoryBudget=1024  PartitionMethod=ROBUST  MultibodyUseLocalSolver=off  MultibodyLocalSolverChoice=ODE1  MultibodyLocalSolverSampleTime=0.001
  Voltage Sensor : fl_lib/Electrical/Electrical Sensors/Voltage Sensor
  Voltage Sensor1 : fl_lib/Electrical/Electrical Sensors/Voltage Sensor
  Voltage Sensor2 : fl_lib/Electrical/Electrical Sensors/Voltage Sensor
  i_fb : Scope  NumInputPorts=2
  iin/uin : Scope  NumInputPorts=2
  iout/uout : Scope  NumInputPorts=2
  opa_raw_mos_2 : Subsystem  mask{u_dd=15, u_ss=-15, Rbias=1e3, Ibias=10e-3}
      mask prompts: u_dd "Udd"; u_ss "Uss"
  opa_raw_mos_with_ibias_clamped : Subsystem  mask{u_dd=15, u_ss=-15, Rbias=1e3, Ibias=1}
      mask prompts: u_dd "Udd"; u_ss "Uss"
  uin_1/uout : Scope  NumInputPorts=2
  uin_2/uout : Scope  NumInputPorts=2
  wires:
  PS-Simulink Converter5/1 -> i_fb/1  "i_fb_2"
  PS-Simulink Converter4/1 -> i_fb/2  "i_fb_1"
  PS-Simulink Converter3/1 -> iin/uin/1  "iin"
  PS-Simulink Converter2/1 -> iout/uout/1  "iout"
  PS-Simulink Converter1/1 -> uin_2/uout/1, iin/uin/2  "uin"
  PS-Simulink Converter/1 -> uin_1/uout/2, uin_2/uout/2, iout/uout/2  "uout"
  Sine Wave/1 -> Simulink-PS Converter/1
  PS-Simulink Converter6/1 -> uin_1/uout/1  "uin"
  connections:
  Controlled Voltage Source/LConn1 -- R4_1/LConn1
  Current Sensor3/RConn1 -- PS-Simulink Converter5/LConn1
  R4_330/RConn1 -- Current Sensor3/LConn1
  PS-Simulink Converter4/LConn1 -- Current Sensor2/RConn1
  Current Sensor2/LConn1 -- R3_330/RConn1
  R5_3R3/RConn1 -- Current Sensor/LConn1 -- Current Sensor2/RConn2 -- Voltage Sensor/LConn1
  R3_330/LConn1 -- opa_raw_mos_with_ibias_clamped/LConn1 -- R1_470/RConn1
  PS-Simulink Converter3/LConn1 -- Current Sensor1/RConn1
  Current Sensor3/RConn2 -- opa_raw_mos_with_ibias_clamped/RConn1 -- R5_3R3/LConn1
  R4_330/LConn1 -- opa_raw_mos_with_ibias_clamped/LConn2 -- R2_470/LConn1
  Rload_5/RConn1 -- opa_raw_mos_with_ibias_clamped/RConn2 -- Voltage Sensor/RConn2
  Electrical Reference1/LConn1 -- Controlled Voltage Source/RConn2 -- Solver Configuration/RConn1
  PS-Simulink Converter/LConn1 -- Voltage Sensor/RConn1
  Electrical Reference7/LConn1 -- R2_470/RConn1
  Simulink-PS Converter/RConn1 -- Controlled Voltage Source/RConn1
  Electrical Reference2/LConn1 -- Voltage Sensor1/RConn2
  R1_470/LConn1 -- Voltage Sensor1/LConn1 -- Current Sensor1/RConn2
  PS-Simulink Converter2/LConn1 -- Current Sensor/RConn1
  Current Sensor/RConn2 -- Rload_5/LConn1
  PS-Simulink Converter1/LConn1 -- Voltage Sensor1/RConn1
  opa_raw_mos_2/LConn1 -- Voltage Sensor2/LConn1 -- R4_1/RConn1
  PS-Simulink Converter6/LConn1 -- Voltage Sensor2/RConn1
  Electrical Reference4/LConn1 -- Voltage Sensor2/RConn2
  opa_raw_mos_2/LConn2 -- Current Sensor1/LConn1 -- opa_raw_mos_2/RConn1
